simulink model "USV_SAR_GNSS"  (R2026b)
settings: Solver=VariableStepAuto  StopTime=600
undefined symbols (not defined in the file): arrival_dwell_time, arrival_radius, arrival_speed, assistance_duration, battery_capacity_J, battery_initial_soc, battery_return_soc, current_bias_x, current_bias_y, current_change_time, current_estimation_tau, current_x, current_y, drag_r, drag_u, F_max, gnss_bias_x, gnss_bias_y, gnss_loss_enabled, gnss_loss_end, gnss_loss_start, gnss_position_sigma, gnss_sample_time, home_x, home_y, inertia_z, initial_heading, initial_x, initial_y, integral_activation_radius, K_aw, K_distance, Kd_heading, Ki_position, Ki_u, Kp_heading, Kp_u, M_max, mass_usv, mob_contact_loss_enabled, mob_contact_loss_end, mob_contact_loss_start, mob_drift_change_enabled, mob_drift_change_time, mob_drift_factor_after, mob_position_sigma, mob_sensor_sample_time, mob_track_alpha, mob_track_beta, mob_track_max_age, mob_track_sample_time, nav_alpha, nav_beta, nav_max_prediction_time, nav_sample_time, num_waypoints, P_aux, P_thrust_max, P_turn_max, position_integral_limit ... (+6)
libraries: simulink x7
(part 1 of 2)
settings Model: Creator=pablo  LastModifiedBy=pablo

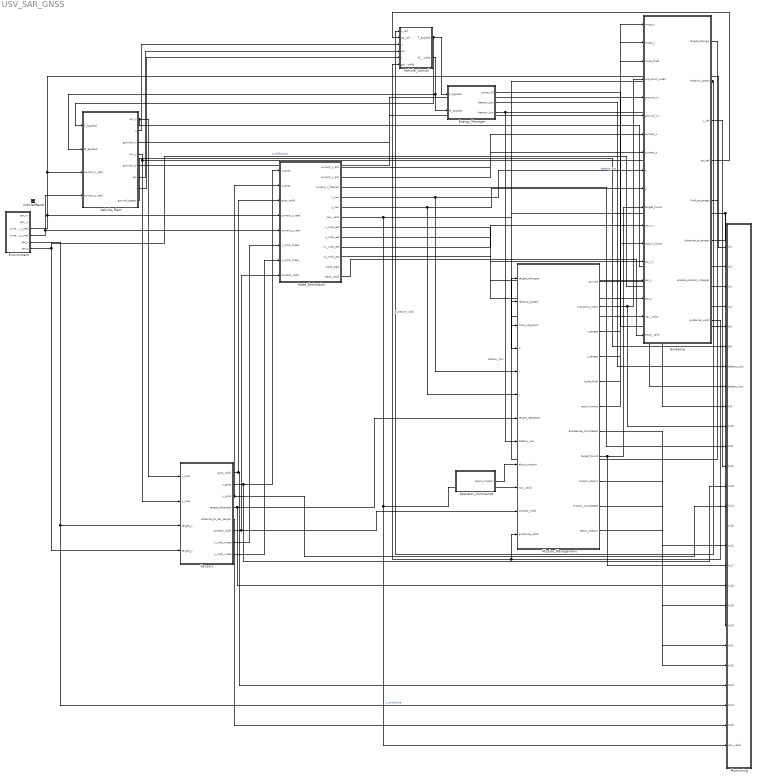
== system USV_SAR_GNSS ==
  Energy_Manager : Subsystem
  Environment : Subsystem
  Guidance : Subsystem
  Mission_Management : Subsystem
  Monitoring : Subsystem
  Operator_Commands : Subsystem
  Sensors : Subsystem
  State_Estimation : Subsystem
  Vehicle_Control : Subsystem
  Vehicle_Plant : Subsystem
  untitledPanel : Subsystem  Tag=HiddenForWebPanel  IsWebBlockPanel=on
  wires:
  Environment/6(sar_y) -> Monitoring/3(In3), Sensors/4(target_y)  "y_mob_true"
  Environment/5(sar_x) -> Monitoring/24(In24), Sensors/3(target_x)  "x_mob_true"
  Environment/4(current_y_real) -> State_Estimation/5(current_y_real), Vehicle_Plant/4(current_y_real)
  Environment/3(current_x_real) -> Monitoring/1(In1), Vehicle_Plant/3(current_x_real), State_Estimation/4(current_x_real)
  Vehicle_Plant/1(usv_x) -> Monitoring/2(In2), Sensors/1(x_true)
  State_Estimation/6(nav_valid) -> Mission_Management/10(nav_valid), Monitoring/26(nav_valid), Guidance/17(nav_valid)
  Vehicle_Plant/2(u) -> Vehicle_Control/3(u)
  Vehicle_Plant/3(ground_vx) -> Guidance/5(ground_vx)
  Vehicle_Plant/4(usv_y) -> Monitoring/4(In4), Sensors/2(y_true)
  Vehicle_Plant/5(ground_vy) -> Guidance/6(ground_vy)
  Vehicle_Plant/6(psi) -> Vehicle_Control/4(psi)
  Energy_Manager/2(battery_soc) -> Monitoring/7(battery_soc)  "battery_soc"
  Vehicle_Plant/7(r) -> Vehicle_Control/5(r)
  Sensors/6(contact_valid) -> Mission_Management/11(contact_valid), State_Estimation/8(contact_valid)
  Vehicle_Plant/8(ground_speed) -> Monitoring/6(In6)
  Sensors/1(gnss_valid) -> Monitoring/23(In23), State_Estimation/3(gnss_valid)
  Operator_Commands/1(abort_mission) -> Mission_Management/9(abort_mission)
  State_Estimation/7(x_mob_est) -> Guidance/15(sar_x)
  Sensors/2(x_gnss) -> Monitoring/13(In13), State_Estimation/1(x_gnss)
  State_Estimation/10(vy_mob_est) -> Guidance/14(sar_vy)
  Sensors/3(y_gnss) -> Monitoring/14(In14), State_Estimation/2(y_gnss)
  State_Estimation/1(current_x_est) -> Guidance/7(current_x)
  Sensors/4(target_detected) -> Monitoring/18(In18), Mission_Management/7(target_detected)
  State_Estimation/4(x_nav) -> Guidance/9(x), Mission_Management/5(x)
  Sensors/5(distance_to_sar_target) -> Monitoring/25(In25)
  Sensors/7(x_mob_meas) -> State_Estimation/6(x_mob_meas)
  Sensors/8(y_mob_meas) -> State_Estimation/7(y_mob_meas)
  State_Estimation/2(current_y_est) -> Guidance/8(current_y)
  State_Estimation/3(current_x_filtered) -> Monitoring/11(In11)
  State_Estimation/5(y_nav) -> Guidance/10(y), Mission_Management/6(y)
  State_Estimation/8(y_mob_est) -> Guidance/16(sar_y)
  State_Estimation/9(vx_mob_est) -> Guidance/12(sar_vx)
  Mission_Management/2(waypoint_index) -> Monitoring/10(In10), Guidance/4(waypoint_index)
  Vehicle_Control/1(F_applied) -> Vehicle_Plant/1(F_applied), Energy_Manager/1(F_applied)
  Vehicle_Control/2(M_applied) -> Vehicle_Plant/2(M_applied), Energy_Manager/2(M_applied)
  Energy_Manager/3(battery_low) -> Monitoring/8(battery_low), Mission_Management/8(battery_low)  "battery_low"
  Energy_Manager/1(power_W) -> Monitoring/5(In5)
  Mission_Management/1(arrived) -> Monitoring/9(In9)
  Mission_Management/3(x_target) -> Guidance/1(route_x)
  Guidance/6(distance_to_target) -> Monitoring/20(In20), Mission_Management/4(d)
  Guidance/2(relative_speed) -> Monitoring/12(In12), Mission_Management/2(relative_speed)
  Mission_Management/4(y_target) -> Guidance/2(route_y)
  Mission_Management/5(route_final) -> Guidance/3(route_final)
  Mission_Management/6(return_home) -> Guidance/13(return_home)
  Mission_Management/7(assistance_completed) -> Monitoring/16(In16)
  Guidance/3(u_ref) -> Vehicle_Control/1(u_ref)
  Mission_Management/8(target_found) -> Monitoring/17(In17), Guidance/11(target_found)
  Mission_Management/9(mission_status) -> Monitoring/19(In19)
  Mission_Management/10(mission_completed) -> Monitoring/21(In21)
  Mission_Management/11(return_reason) -> Monitoring/22(In22)
  Guidance/5(hold_at_target) -> Mission_Management/3(final_waypoint)
  Guidance/1(target_change) -> Mission_Management/1(target_changed)
  Guidance/4(psi_ref) -> Vehicle_Control/2(psi_ref)
  State_Estimation/12(track_valid) -> Guidance/18(track_valid)
  Guidance/8(guidance_valid) -> Mission_Management/12(guidance_valid), Vehicle_Control/6(guidance_valid)  "guidance_valid"

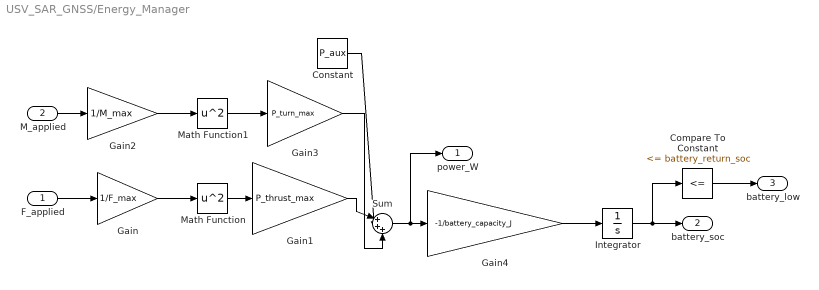
== system USV_SAR_GNSS/Energy_Manager ==
  F_applied : Inport
  M_applied : Inport  Port=2
  Compare To Constant : simulink/Logic and Bit Operations/Compare To Constant  relop=<=  const=battery_return_soc  OutDataTypeStr=boolean
  Constant : Constant  Value=P_aux
  Gain : Gain  Gain=1/F_max
  Gain1 : Gain  Gain=P_thrust_max
  Gain2 : Gain  Gain=1/M_max
  Gain3 : Gain  Gain=P_turn_max
  Gain4 : Gain  Gain=-1/battery_capacity_J
  Integrator : Integrator  InitialCondition=battery_initial_soc  LimitOutput=on  UpperSaturationLimit=1  LowerSaturationLimit=0
  Math Function : Math  Operator=square
  Math Function1 : Math  Operator=square
  Sum : Sum  Inputs=|+++
  power_W : Outport
  battery_soc : Outport  Port=2
  battery_low : Outport  Port=3
  wires:
  Gain2/1 -> Math Function1/1
  M_applied/1 -> Gain2/1
  F_applied/1 -> Gain/1
  Math Function1/1 -> Gain3/1
  Gain/1 -> Math Function/1
  Math Function/1 -> Gain1/1
  Constant/1 -> Sum/2
  Gain3/1 -> Sum/3
  Gain1/1 -> Sum/1
  Sum/1 -> power_W/1, Gain4/1
  Gain4/1 -> Integrator/1
  Integrator/1 -> battery_soc/1, Compare To Constant/1
  Compare To Constant/1 -> battery_low/1

== system USV_SAR_GNSS/Environment ==
  Current_Environment : Subsystem
  SAR_Target_Motion : Subsystem
  sar_vx : Outport
  sar_vy : Outport  Port=2
  current_x_real : Outport  Port=3
  current_y_real : Outport  Port=4
  sar_x : Outport  Port=5
  sar_y : Outport  Port=6
  wires:
  Current_Environment/2(current_y_real) -> SAR_Target_Motion/2(current_y_real), current_y_real/1
  Current_Environment/1(current_x_real) -> current_x_real/1, SAR_Target_Motion/1(current_x_real)
  SAR_Target_Motion/3(sar_vx) -> sar_vx/1  "vx_mob_true"
  SAR_Target_Motion/1(sar_x) -> sar_x/1
  SAR_Target_Motion/4(sar_vy) -> sar_vy/1  "vy_mob_true"
  SAR_Target_Motion/2(sar_y) -> sar_y/1

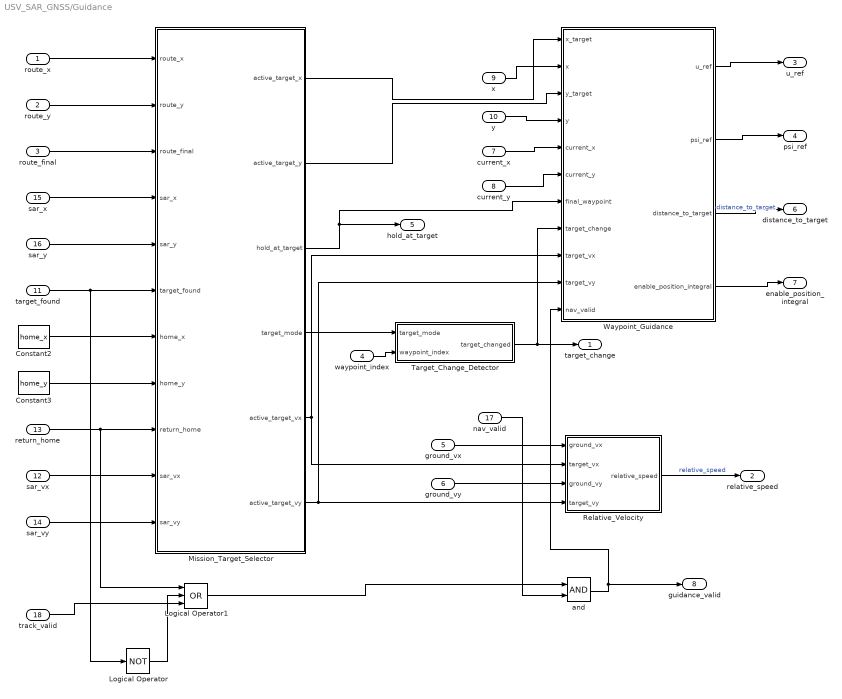
== system USV_SAR_GNSS/Guidance ==
  route_x : Inport
  route_y : Inport  Port=2
  route_final : Inport  Port=3
  waypoint_index : Inport  Port=4
  ground_vx : Inport  Port=5
  ground_vy : Inport  Port=6
  current_x : Inport  Port=7
  current_y : Inport  Port=8
  x : Inport  Port=9
  y : Inport  Port=10
  target_found : Inport  Port=11
  sar_vx : Inport  Port=12
  return_home : Inport  Port=13
  sar_vy : Inport  Port=14
  sar_x : Inport  Port=15
  sar_y : Inport  Port=16
  nav_valid : Inport  Port=17
  track_valid : Inport  Port=18
  Constant2 : Constant  Value=home_x
  Constant3 : Constant  Value=home_y
  Logical Operator : Logic  Operator=NOT  AllPortsSameDT=off  OutDataTypeStr=boolean
  Logical Operator1 : Logic  Operator=OR  Inputs=3  AllPortsSameDT=off  OutDataTypeStr=boolean
  Mission_Target_Selector : Subsystem
  Relative_Velocity : Subsystem
  Target_Change_Detector : Subsystem
  Waypoint_Guidance : Subsystem
  and : Logic  AllPortsSameDT=off  OutDataTypeStr=boolean
  target_change : Outport
  relative_speed : Outport  Port=2
  u_ref : Outport  Port=3
  psi_ref : Outport  Port=4
  hold_at_target : Outport  Port=5
  distance_to_target : Outport  Port=6
  enable_position_integral : Outport  Port=7
  guidance_valid : Outport  Port=8
  wires:
  Waypoint_Guidance/1(u_ref) -> u_ref/1
  Constant3/1 -> Mission_Target_Selector/8(home_y)
  ground_vx/1 -> Relative_Velocity/1(ground_vx)
  Constant2/1 -> Mission_Target_Selector/7(home_x)
  Waypoint_Guidance/3(distance_to_target) -> distance_to_target/1  "distance_to_target"
  Relative_Velocity/1(relative_speed) -> relative_speed/1  "relative_speed"
  route_x/1 -> Mission_Target_Selector/1(route_x)
  route_y/1 -> Mission_Target_Selector/2(route_y)
  Waypoint_Guidance/2(psi_ref) -> psi_ref/1
  target_found/1 -> Logical Operator/1, Mission_Target_Selector/6(target_found)
  sar_x/1 -> Mission_Target_Selector/4(sar_x)
  route_final/1 -> Mission_Target_Selector/3(route_final)
  sar_y/1 -> Mission_Target_Selector/5(sar_y)
  return_home/1 -> Logical Operator1/1, Mission_Target_Selector/9(return_home)
  sar_vx/1 -> Mission_Target_Selector/10(sar_vx)
  Mission_Target_Selector/1(active_target_x) -> Waypoint_Guidance/1(x_target)
  sar_vy/1 -> Mission_Target_Selector/11(sar_vy)
  ground_vy/1 -> Relative_Velocity/3(ground_vy)
  y/1 -> Waypoint_Guidance/4(y)
  Mission_Target_Selector/2(active_target_y) -> Waypoint_Guidance/3(y_target)
  Mission_Target_Selector/3(hold_at_target) -> Waypoint_Guidance/7(final_waypoint), hold_at_target/1
  Mission_Target_Selector/4(target_mode) -> Target_Change_Detector/1(target_mode)
  Mission_Target_Selector/5(active_target_vx) -> Waypoint_Guidance/9(target_vx), Relative_Velocity/2(target_vx)
  Mission_Target_Selector/6(active_target_vy) -> Waypoint_Guidance/10(target_vy), Relative_Velocity/4(target_vy)
  waypoint_index/1 -> Target_Change_Detector/2(waypoint_index)
  x/1 -> Waypoint_Guidance/2(x)
  Waypoint_Guidance/4(enable_position_integral) -> enable_position_integral/1
  current_x/1 -> Waypoint_Guidance/5(current_x)
  current_y/1 -> Waypoint_Guidance/6(current_y)
  Target_Change_Detector/1(target_changed) -> Waypoint_Guidance/8(target_change), target_change/1
  nav_valid/1 -> and/2
  track_valid/1 -> Logical Operator1/3
  Logical Operator/1 -> Logical Operator1/2
  Logical Operator1/1 -> and/1
  and/1 -> Waypoint_Guidance/11(nav_valid), guidance_valid/1

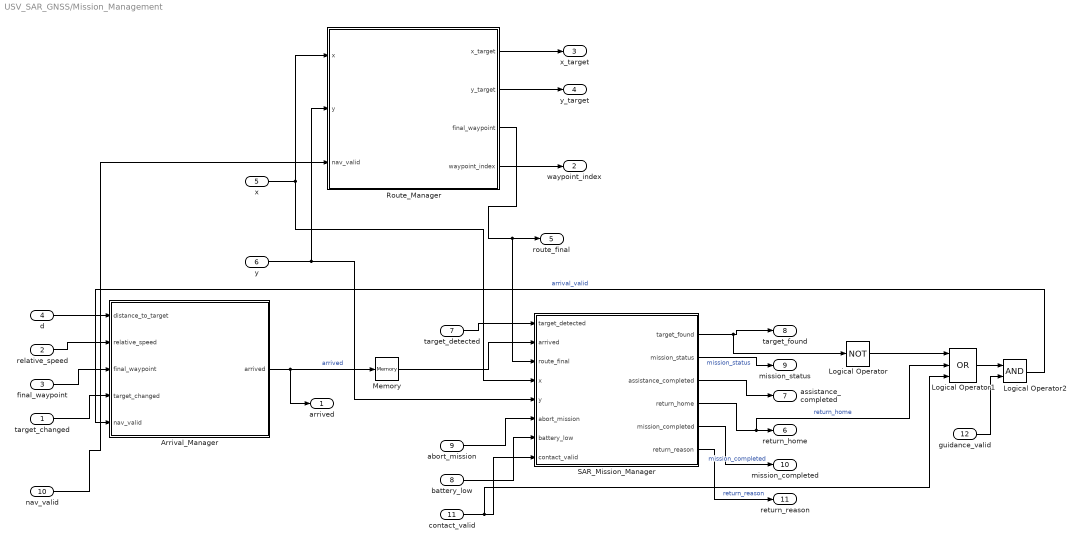
== system USV_SAR_GNSS/Mission_Management ==
  target_changed : Inport
  relative_speed : Inport  Port=2
  final_waypoint : Inport  Port=3
  d : Inport  Port=4
  x : Inport  Port=5
  y : Inport  Port=6
  target_detected : Inport  Port=7
  battery_low : Inport  Port=8
  abort_mission : Inport  Port=9
  nav_valid : Inport  Port=10
  contact_valid : Inport  Port=11
  guidance_valid : Inport  Port=12
  Arrival_Manager : Stateflow chart  TreatAsAtomicUnit=on
  Logical Operator : Logic  Operator=NOT  AllPortsSameDT=off  OutDataTypeStr=boolean
  Logical Operator1 : Logic  Operator=OR  Inputs=3  AllPortsSameDT=off  OutDataTypeStr=boolean
  Logical Operator2 : Logic  AllPortsSameDT=off  OutDataTypeStr=boolean
  Memory : Memory
  Route_Manager : Stateflow chart  TreatAsAtomicUnit=on
  SAR_Mission_Manager : Stateflow chart  TreatAsAtomicUnit=on
  arrived : Outport
  waypoint_index : Outport  Port=2
  x_target : Outport  Port=3
  y_target : Outport  Port=4
  route_final : Outport  Port=5
  return_home : Outport  Port=6
  assistance_completed : Outport  Port=7
  target_found : Outport  Port=8
  mission_status : Outport  Port=9
  mission_completed : Outport  Port=10
  return_reason : Outport  Port=11
  wires:
  d/1 -> Arrival_Manager/1(distance_to_target)
  SAR_Mission_Manager/6(return_reason) -> return_reason/1  "return_reason"
  target_changed/1 -> Arrival_Manager/4(target_changed)
  final_waypoint/1 -> Arrival_Manager/3(final_waypoint)
  SAR_Mission_Manager/3(assistance_completed) -> assistance_completed/1
  abort_mission/1 -> SAR_Mission_Manager/6(abort_mission)
  relative_speed/1 -> Arrival_Manager/2(relative_speed)
  Arrival_Manager/1(arrived) -> arrived/1, Memory/1  "arrived"
  y/1 -> SAR_Mission_Manager/5(y), Route_Manager/2(y)
  x/1 -> SAR_Mission_Manager/4(x), Route_Manager/1(x)
  Route_Manager/1(x_target) -> x_target/1
  Route_Manager/2(y_target) -> y_target/1
  Route_Manager/3(final_waypoint) -> SAR_Mission_Manager/3(route_final), route_final/1
  Route_Manager/4(waypoint_index) -> waypoint_index/1
  target_detected/1 -> SAR_Mission_Manager/1(target_detected)
  Memory/1 -> SAR_Mission_Manager/2(arrived)
  battery_low/1 -> SAR_Mission_Manager/7(battery_low)
  SAR_Mission_Manager/1(target_found) -> Logical Operator/1, target_found/1
  SAR_Mission_Manager/2(mission_status) -> mission_status/1  "mission_status"
  SAR_Mission_Manager/4(return_home) -> Logical Operator1/2, return_home/1  "return_home"
  SAR_Mission_Manager/5(mission_completed) -> mission_completed/1  "mission_completed"
  nav_valid/1 -> Route_Manager/3(nav_valid)
  contact_valid/1 -> Logical Operator1/3, SAR_Mission_Manager/8(contact_valid)
  Logical Operator/1 -> Logical Operator1/1
  Logical Operator1/1 -> Logical Operator2/1
  guidance_valid/1 -> Logical Operator2/2
  Logical Operator2/1 -> Arrival_Manager/5(nav_valid)  "arrival_valid"

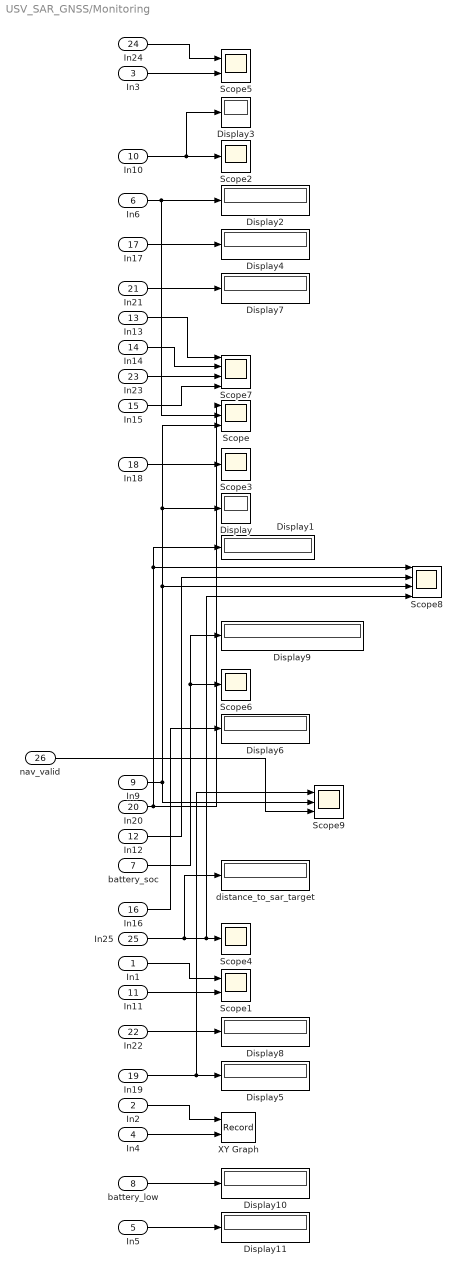
== system USV_SAR_GNSS/Monitoring ==
  In1 : Inport
  In2 : Inport  Port=2
  In3 : Inport  Port=3
  In4 : Inport  Port=4
  In5 : Inport  Port=5
  In6 : Inport  Port=6
  battery_soc : Inport  Port=7
  battery_low : Inport  Port=8
  In9 : Inport  Port=9
  In10 : Inport  Port=10
  In11 : Inport  Port=11
  In12 : Inport  Port=12
  In13 : Inport  Port=13
  In14 : Inport  Port=14
  In15 : Inport  Port=15
  In16 : Inport  Port=16
  In17 : Inport  Port=17
  In18 : Inport  Port=18
  In19 : Inport  Port=19
  In20 : Inport  Port=20
  In21 : Inport  Port=21
  In22 : Inport  Port=22
  In23 : Inport  Port=23
  In24 : Inport  Port=24
  In25 : Inport  Port=25
  nav_valid : Inport  Port=26
  Display{,1..11} (12 alike) : Display
  Scope : Scope  NumInputPorts=3
      settings: ActiveDisplayYMinimum=-3.9141031212329302  ActiveDisplayYMaximum=39.009126348576444
  Scope1 : Scope  NumInputPorts=2
      settings: ActiveDisplayYMinimum=-0.25  ActiveDisplayYMaximum=0.25
  Scope{2..4,6} (4 alike) : Scope
      Scope2 settings: ActiveDisplayYMinimum=-8.8280515458215767  ActiveDisplayYMaximum=9.3125380233394175  DataLoggingVariableName=ScopeData2
      Scope3 settings: ActiveDisplayYMinimum=0.096949603045415472  ActiveDisplayYMaximum=1.0318774717483707  DataLoggingVariableName=ScopeData3
      Scope4 settings: ActiveDisplayYMinimum=-1.9004946435428702E+6  ActiveDisplayYMaximum=1.5322246928084393E+6  DataLoggingVariableName=ScopeData4
      Scope6 settings: ActiveDisplayYMinimum=0.9  ActiveDisplayYMaximum=1.1  DataLoggingVariableName=ScopeData6
  Scope5 : Scope  NumInputPorts=2
      settings: ActiveDisplayYMinimum=-44.000000000000014  ActiveDisplayYMaximum=76.000000000000028  DataLoggingVariableName=ScopeData5
  Scope7 : Scope  NumInputPorts=4
      settings: ActiveDisplayYMinimum=-12.806626439493318  ActiveDisplayYMaximum=22.267972808748297  DataLoggingVariableName=ScopeData7
  Scope8 : Scope  NumInputPorts=4
      settings: ActiveDisplayYMinimum=-3.0987987776116084  ActiveDisplayYMaximum=12.732026530654965  DataLoggingVariableName=ScopeData8
  Scope9 : Scope  NumInputPorts=3
      settings: ActiveDisplayYMinimum=-0.62499999999999989  ActiveDisplayYMaximum=5.625  DataLoggingVariableName=ScopeData9
  XY Graph : Record  NumPorts=2.0  FileSettingsInternal="{\"entries\":[{\"content\":{\"excelSettings\":{\"content\":{},\"type\":\"Streamout.ExcelSettings\"},\"parquetSettings\":{\"content\":{},\"type\":\"Streamout.ParquetSettings\"}},\"type\":\"Streamout.FileSettingStorage\",\"uuid\":\"\"}],\"packageUris\":[\"http:\\/\\/schema.mathworks.com\\/mf0\\/streamout_blocks\\/R2020a\"],\"version\":\"1.0\"}"  FrameSettings=[0, 0]  Layout=[1 1]  SignalsInternal="{\"entries\":[{\"content\":{\"signals\":[{\"content\":{\"blockPath\":[],\"dimensions\":[1],\"domain\":\"\",\"lineColor\":\"#7e2f8e\",\"lineWidth\":2,\"plots\":[ 1 ],\"port\":1,\"sid\":[\"\"],\"signalID\":1,\"signalName\":\"In2\"},\"type\":\"RecordBlkView.Signal\",\"uuid\":\"\"},{\"content\":{\"blockPath\":[],\"dimensions\":[1],\"domain\":\"\",\"lineColor\":\"#77ac30\",\"lineWidth\":2,\"plots\":[ 1 ],\"port\":2,\"sid\":[\"\"],\"signalID\":2,\"signalName\":\"In4\"},\"type\":\"RecordBlkView.Signal\",\"uuid\":\"\"}]},\"type\":\"RecordBlkView.InputSignals\",\"uuid\":\"\"}],\"packageUris\":[\"http:\\/\\/schema.mathworks.com\\/mf0\\/streamout_blocks\\/R2020a\"],\"version\":\"1.0\"}"  VisualizationBindings="{\"xyplotplugin\":{\"info\":[{\"series\":[{\"bindingParametersList\":[{\"parameter\":\"X-Axis\",\"signalID\":1,\"signalName\":\"In2\"},{\"parameter\":\"Y-Axis\",\"signalID\":2,\"signalName\":\"In4\"}],\"seriesID\":0}],\"subplotID\":1}]}}"  CompatibilityTag=XY
  distance_to_sar_target : Display
  wires:
  In22/1 -> Display8/1
  In6/1 -> Scope/2, Display2/1
  In14/1 -> Scope7/2
  In5/1 -> Display11/1
  In21/1 -> Display7/1
  In13/1 -> Scope7/1
  In1/1 -> Scope1/1
  In25/1 -> Scope8/4, Scope4/1, distance_to_sar_target/1
  In9/1 -> Display/1, Scope/3, Scope8/3, Scope9/2
  In17/1 -> Display4/1
  In2/1 -> XY Graph/1
  In18/1 -> Scope3/1
  In10/1 -> Scope2/1, Display3/1
  In19/1 -> Scope9/1, Display5/1
  In11/1 -> Scope1/2
  In3/1 -> Scope5/2
  battery_low/1 -> Display10/1
  In16/1 -> Display6/1
  In24/1 -> Scope5/1
  battery_soc/1 -> Display9/1, Scope6/1
  In15/1 -> Scope7/4
  In23/1 -> Scope7/3
  In4/1 -> XY Graph/2
  In12/1 -> Scope8/2
  In20/1 -> Display1/1, Scope8/1, Scope/1
  nav_valid/1 -> Scope9/3

== system USV_SAR_GNSS/Operator_Commands ==
  Cancel_Release_Step : Step  Time=11  FinalValue=0  SampleTime=0
  Data Type Conversion : DataTypeConversion  OutDataTypeStr=boolean  SaturateOnIntegerOverflow=off  RndMeth=Floor
  Step : Step  Time=100  FinalValue=0  SampleTime=0
  Sum : Sum  Inputs=|+-
  abort_mission : Outport
  wires:
  Step/1 -> Sum/1
  Data Type Conversion/1 -> abort_mission/1  "abort_mission"
  Sum/1 -> Data Type Conversion/1
  Cancel_Release_Step/1 -> Sum/2

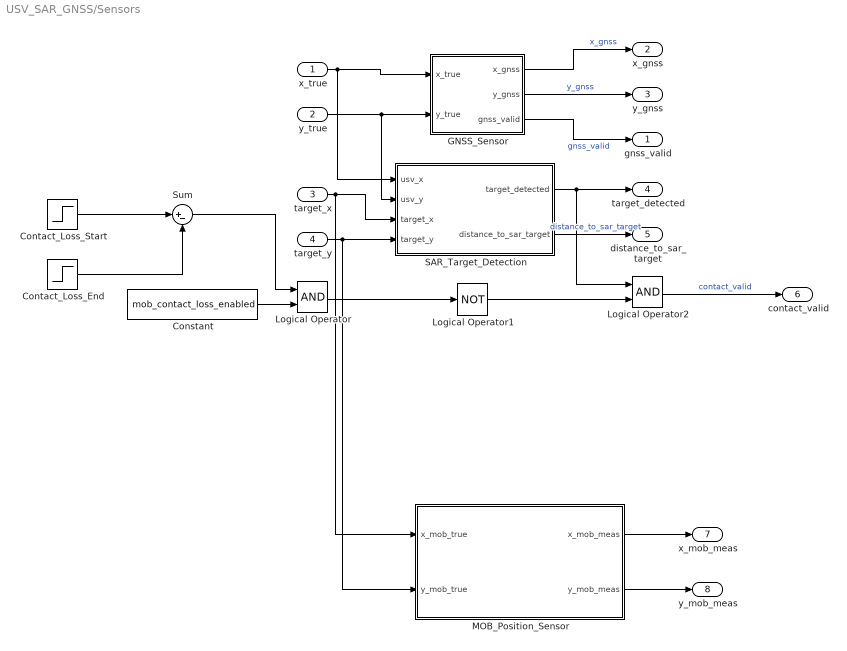
== system USV_SAR_GNSS/Sensors ==
  x_true : Inport
  y_true : Inport  Port=2
  target_x : Inport  Port=3
  target_y : Inport  Port=4
  Constant : Constant  Value=mob_contact_loss_enabled
  Contact_Loss_End : Step  Time=mob_contact_loss_end  SampleTime=0
  Contact_Loss_Start : Step  Time=mob_contact_loss_start  SampleTime=0
  GNSS_Sensor : Subsystem
  Logical Operator : Logic  AllPortsSameDT=off  OutDataTypeStr=boolean
  Logical Operator1 : Logic  Operator=NOT  AllPortsSameDT=off  OutDataTypeStr=boolean
  Logical Operator2 : Logic  AllPortsSameDT=off  OutDataTypeStr=boolean
  MOB_Position_Sensor : Subsystem
  SAR_Target_Detection : Subsystem
  Sum : Sum  Inputs=|+-
  gnss_valid : Outport
  x_gnss : Outport  Port=2
  y_gnss : Outport  Port=3
  target_detected : Outport  Port=4
  distance_to_sar_target : Outport  Port=5
  contact_valid : Outport  Port=6
  x_mob_meas : Outport  Port=7
  y_mob_meas : Outport  Port=8
  wires:
  Constant/1 -> Logical Operator/2
  Sum/1 -> Logical Operator/1
  Contact_Loss_End/1 -> Sum/2
  Contact_Loss_Start/1 -> Sum/1
  target_y/1 -> MOB_Position_Sensor/2(y_mob_true), SAR_Target_Detection/4(target_y)
  target_x/1 -> MOB_Position_Sensor/1(x_mob_true), SAR_Target_Detection/3(target_x)
  y_true/1 -> GNSS_Sensor/2(y_true), SAR_Target_Detection/2(usv_y)
  x_true/1 -> GNSS_Sensor/1(x_true), SAR_Target_Detection/1(usv_x)
  Logical Operator/1 -> Logical Operator1/1
  GNSS_Sensor/1(x_gnss) -> x_gnss/1  "x_gnss"
  GNSS_Sensor/2(y_gnss) -> y_gnss/1  "y_gnss"
  Logical Operator1/1 -> Logical Operator2/2
  GNSS_Sensor/3(gnss_valid) -> gnss_valid/1  "gnss_valid"
  SAR_Target_Detection/1(target_detected) -> Logical Operator2/1, target_detected/1
  SAR_Target_Detection/2(distance_to_sar_target) -> distance_to_sar_target/1  "distance_to_sar_target"
  Logical Operator2/1 -> contact_valid/1  "contact_valid"
  MOB_Position_Sensor/1(x_mob_meas) -> x_mob_meas/1
  MOB_Position_Sensor/2(y_mob_meas) -> y_mob_meas/1

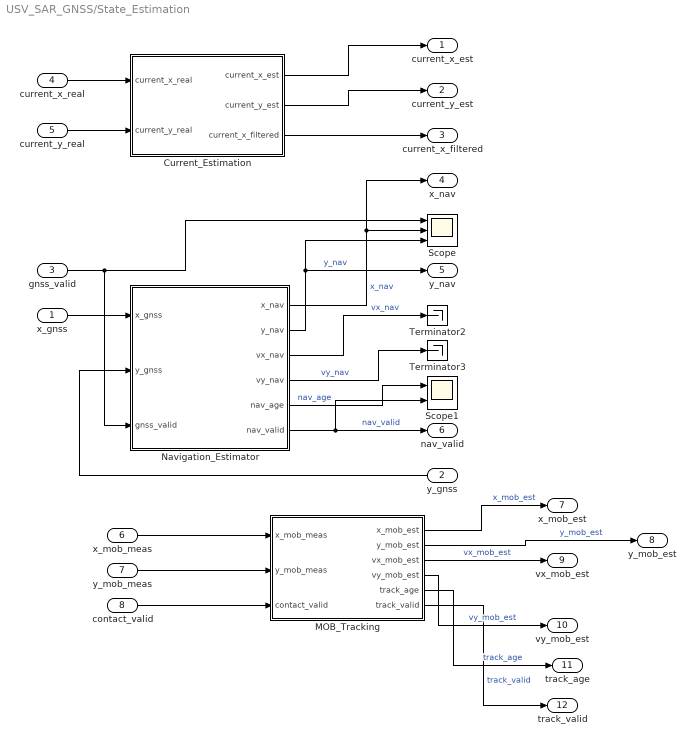
== system USV_SAR_GNSS/State_Estimation ==
  x_gnss : Inport
  y_gnss : Inport  Port=2
  gnss_valid : Inport  Port=3
  current_x_real : Inport  Port=4
  current_y_real : Inport  Port=5
  x_mob_meas : Inport  Port=6
  y_mob_meas : Inport  Port=7
  contact_valid : Inport  Port=8
  Current_Estimation : Subsystem
  MOB_Tracking : Subsystem
  Navigation_Estimator : Subsystem
  Scope : Scope  NumInputPorts=3
      settings: ActiveDisplayYMinimum=-0.26944529643328874  ActiveDisplayYMaximum=48.836838243913448  DataLoggingVariableName=ScopeData10
  Scope1 : Scope  NumInputPorts=2
      settings: ActiveDisplayYMinimum=-2.6125000000000029  ActiveDisplayYMaximum=23.512500000000031  DataLoggingVariableName=ScopeData11
  Terminator2 : Terminator
  Terminator3 : Terminator
  current_x_est : Outport
  current_y_est : Outport  Port=2
  current_x_filtered : Outport  Port=3
  x_nav : Outport  Port=4
  y_nav : Outport  Port=5
  nav_valid : Outport  Port=6
  x_mob_est : Outport  Port=7
  y_mob_est : Outport  Port=8
  vx_mob_est : Outport  Port=9
  vy_mob_est : Outport  Port=10
  track_age : Outport  Port=11
  track_valid : Outport  Port=12
  wires:
  x_gnss/1 -> Navigation_Estimator/1(x_gnss)
  current_x_real/1 -> Current_Estimation/1(current_x_real)
  Current_Estimation/3(current_x_filtered) -> current_x_filtered/1
  Current_Estimation/1(current_x_est) -> current_x_est/1
  gnss_valid/1 -> Scope/1, Navigation_Estimator/3(gnss_valid)
  current_y_real/1 -> Current_Estimation/2(current_y_real)
  Current_Estimation/2(current_y_est) -> current_y_est/1
  Navigation_Estimator/1(x_nav) -> Scope/2, x_nav/1  "x_nav"
  Navigation_Estimator/2(y_nav) -> Scope/3, y_nav/1  "y_nav"
  Navigation_Estimator/3(vx_nav) -> Terminator2/1  "vx_nav"
  Navigation_Estimator/4(vy_nav) -> Terminator3/1  "vy_nav"
  Navigation_Estimator/5(nav_age) -> Scope1/1  "nav_age"
  Navigation_Estimator/6(nav_valid) -> nav_valid/1, Scope1/2  "nav_valid"
  y_gnss/1 -> Navigation_Estimator/2(y_gnss)
  x_mob_meas/1 -> MOB_Tracking/1(x_mob_meas)
  contact_valid/1 -> MOB_Tracking/3(contact_valid)
  y_mob_meas/1 -> MOB_Tracking/2(y_mob_meas)
  MOB_Tracking/1(x_mob_est) -> x_mob_est/1  "x_mob_est"
  MOB_Tracking/2(y_mob_est) -> y_mob_est/1  "y_mob_est"
  MOB_Tracking/3(vx_mob_est) -> vx_mob_est/1  "vx_mob_est"
  MOB_Tracking/4(vy_mob_est) -> vy_mob_est/1  "vy_mob_est"
  MOB_Tracking/5(track_age) -> track_age/1  "track_age"
  MOB_Tracking/6(track_valid) -> track_valid/1  "track_valid"

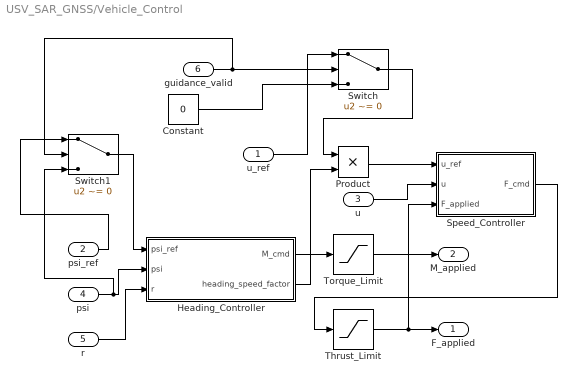
== system USV_SAR_GNSS/Vehicle_Control ==
  u_ref : Inport
  psi_ref : Inport  Port=2
  u : Inport  Port=3
  psi : Inport  Port=4
  r : Inport  Port=5
  guidance_valid : Inport  Port=6
  Constant : Constant  Value=0
  Heading_Controller : Subsystem
  Product : Product
  Speed_Controller : Subsystem
  Switch : Switch  Criteria=u2 ~= 0  SaturateOnIntegerOverflow=off  InputSameDT=off
  Switch1 : Switch  Criteria=u2 ~= 0  SaturateOnIntegerOverflow=off  InputSameDT=off
  Thrust_Limit : Saturate  UpperLimit=F_max  LowerLimit=-F_max
  Torque_Limit : Saturate  UpperLimit=M_max  LowerLimit=-M_max
  F_applied : Outport
  M_applied : Outport  Port=2
  wires:
  psi_ref/1 -> Switch1/1
  psi/1 -> Switch1/3, Heading_Controller/2(psi)
  Heading_Controller/2(heading_speed_factor) -> Product/2
  Product/1 -> Speed_Controller/1(u_ref)
  Heading_Controller/1(M_cmd) -> Torque_Limit/1
  u_ref/1 -> Switch/1
  r/1 -> Heading_Controller/3(r)
  u/1 -> Speed_Controller/2(u)
  Torque_Limit/1 -> M_applied/1
  Thrust_Limit/1 -> Speed_Controller/3(F_applied), F_applied/1
  Speed_Controller/1(F_cmd) -> Thrust_Limit/1
  guidance_valid/1 -> Switch1/2, Switch/2
  Constant/1 -> Switch/3
  Switch/1 -> Product/1
  Switch1/1 -> Heading_Controller/1(psi_ref)

== system USV_SAR_GNSS/Vehicle_Plant ==
  F_applied : Inport
  M_applied : Inport  Port=2
  current_x_real : Inport  Port=3
  current_y_real : Inport  Port=4
  USV_Dynamics : Subsystem
  USV_Kinematics : Subsystem
  usv_x : Outport
  u : Outport  Port=2
  ground_vx : Outport  Port=3
  usv_y : Outport  Port=4
  ground_vy : Outport  Port=5
  psi : Outport  Port=6
  r : Outport  Port=7
  ground_speed : Outport  Port=8
  wires:
  USV_Kinematics/2(y) -> usv_y/1  "usv_y"
  F_applied/1 -> USV_Dynamics/1(F_cmd)
  M_applied/1 -> USV_Dynamics/2(M_cmd)
  USV_Dynamics/1(u) -> USV_Kinematics/1(u), u/1
  USV_Dynamics/2(r) -> r/1, USV_Kinematics/2(r)
  USV_Kinematics/1(x) -> usv_x/1  "usv_x"
  current_x_real/1 -> USV_Kinematics/3(current_x)
  current_y_real/1 -> USV_Kinematics/4(current_y)
  USV_Kinematics/3(psi) -> psi/1
  USV_Kinematics/4(ground_speed) -> ground_speed/1
  USV_Kinematics/5(ground_vx) -> ground_vx/1
  USV_Kinematics/6(ground_vy) -> ground_vy/1

== system USV_SAR_GNSS/untitledPanel ==
  Display12 : DisplayBlock  Tag=HiddenForWebPanel  PanelInfo="{\"height\":39,\"left\":17,\"panelId\":\"panelId-7d76bbda-0191-40eb-92e3-69925966ccdc\",\"top\":17,\"type\":\"panelChild\",\"version\":\"2019b\",\"width\":174,\"zIndex\":1500002}"  LabelPosition=Hide  Transparency=1  GridColor=[0.502, 0.502, 0.502]
  Display13 : DisplayBlock  Tag=HiddenForWebPanel  PanelInfo="{\"height\":39,\"left\":16,\"panelId\":\"panelId-7d76bbda-0191-40eb-92e3-69925966ccdc\",\"top\":70,\"type\":\"panelChild\",\"version\":\"2019b\",\"width\":174,\"zIndex\":1500004}"  LabelPosition=Hide  Transparency=1  GridColor=[0.502, 0.502, 0.502]
  Display14 : DisplayBlock  Tag=HiddenForWebPanel  PanelInfo="{\"height\":39,\"left\":16,\"panelId\":\"panelId-7d76bbda-0191-40eb-92e3-69925966ccdc\",\"top\":119,\"type\":\"panelChild\",\"version\":\"2019b\",\"width\":174,\"zIndex\":1500006}"  LabelPosition=Hide  Transparency=1  GridColor=[0.502, 0.502, 0.502]
  panelInfo : PanelWebBlock  Tag=HiddenForWebPanel  PanelInfo="{\"compacted\":false,\"height\":256,\"isActiveTab\":true,\"left\":1302,\"name\":\"Panel\",\"panelId\":\"panelId-7d76bbda-0191-40eb-92e3-69925966ccdc\",\"tabIndex\":0,\"tabbedSetId\":\"tabbedSet4358925779\",\"top\":159,\"type\":\"panel\",\"version\":\"2019b\",\"visible\":true,\"width\":237,\"zIndex\":1500002}"  PanelSnapshot=<binary blob, 1920 chars, not shown>

== system USV_SAR_GNSS/Environment/Current_Environment ==
  Step : Step  Time=current_change_time  InitialValue=current_x  FinalValue=current_x_after  SampleTime=0
  Step1 : Step  Time=current_change_time  InitialValue=current_y  FinalValue=current_y_after  SampleTime=0
  current_x_real : Outport
  current_y_real : Outport  Port=2
  wires:
  Step/1 -> current_x_real/1
  Step1/1 -> current_y_real/1

== system USV_SAR_GNSS/Environment/SAR_Target_Motion ==
  current_x_real : Inport
  current_y_real : Inport  Port=2
  Integrator : Integrator  InitialCondition=sar_target_x
  Integrator1 : Integrator  InitialCondition=sar_target_y
  Product : Product
  Product1 : Product
  Step : Step  Time=mob_drift_change_time  InitialValue=sar_drift_factor  FinalValue=sar_drift_factor + double(mob_drift_change_enabled)*(mob_drift_factor_after - sar_drift_factor)  SampleTime=0
  sar_x : Outport
  sar_y : Outport  Port=2
  sar_vx : Outport  Port=3
  sar_vy : Outport  Port=4
  wires:
  Integrator1/1 -> sar_y/1
  Integrator/1 -> sar_x/1
  current_y_real/1 -> Product1/1
  current_x_real/1 -> Product/1
  Product1/1 -> sar_vy/1, Integrator1/1
  Step/1 -> Product/2, Product1/2
  Product/1 -> sar_vx/1, Integrator/1

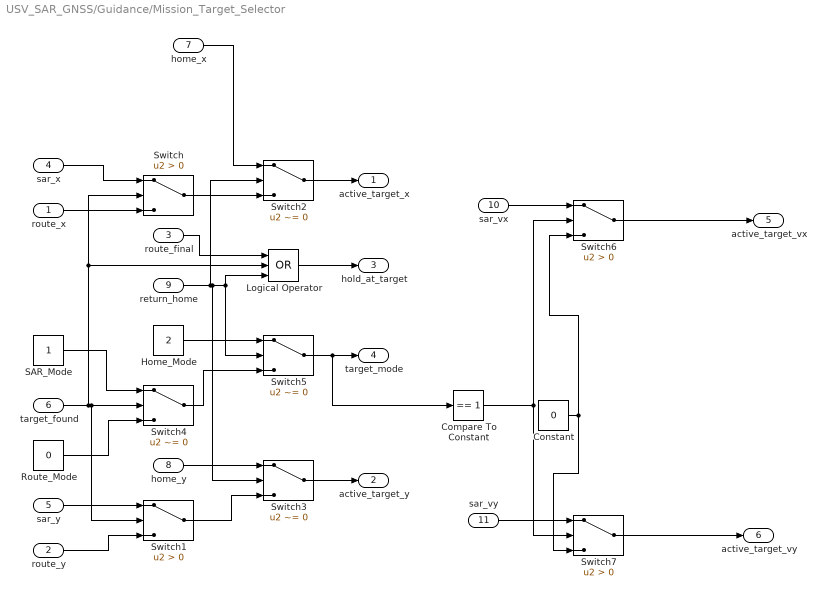
== system USV_SAR_GNSS/Guidance/Mission_Target_Selector ==
  route_x : Inport
  route_y : Inport  Port=2
  route_final : Inport  Port=3
  sar_x : Inport  Port=4
  sar_y : Inport  Port=5
  target_found : Inport  Port=6
  home_x : Inport  Port=7
  home_y : Inport  Port=8
  return_home : Inport  Port=9
  sar_vx : Inport  Port=10
  sar_vy : Inport  Port=11
  Compare To Constant : simulink/Logic and Bit Operations/Compare To Constant  relop===  const=1  OutDataTypeStr=boolean
  Constant : Constant  Value=0
  Home_Mode : Constant  Value=2
  Logical Operator : Logic  Operator=OR  Inputs=3  AllPortsSameDT=off  OutDataTypeStr=boolean
  Route_Mode : Constant  Value=0
  SAR_Mode : Constant
  Switch{,1,6..7} (4 alike) : Switch  Criteria=u2 > Threshold  SaturateOnIntegerOverflow=off  InputSameDT=off
  Switch{2..5} (4 alike) : Switch  Criteria=u2 ~= 0  SaturateOnIntegerOverflow=off  InputSameDT=off
  active_target_x : Outport
  active_target_y : Outport  Port=2
  hold_at_target : Outport  Port=3
  target_mode : Outport  Port=4
  active_target_vx : Outport  Port=5
  active_target_vy : Outport  Port=6
  wires:
  route_final/1 -> Logical Operator/1
  home_x/1 -> Switch2/1
  target_found/1 -> Switch1/2, Switch4/2, Logical Operator/2, Switch/2
  route_y/1 -> Switch1/3
  route_x/1 -> Switch/3
  sar_y/1 -> Switch1/1
  home_y/1 -> Switch3/1
  sar_x/1 -> Switch/1
  Switch4/1 -> Switch5/3
  Route_Mode/1 -> Switch4/3
  SAR_Mode/1 -> Switch4/1
  Switch/1 -> Switch2/3
  return_home/1 -> Logical Operator/3, Switch5/2, Switch3/2, Switch2/2
  Home_Mode/1 -> Switch5/1
  Switch1/1 -> Switch3/3
  Logical Operator/1 -> hold_at_target/1
  Switch2/1 -> active_target_x/1
  Switch5/1 -> Compare To Constant/1, target_mode/1
  Switch3/1 -> active_target_y/1
  Compare To Constant/1 -> Switch6/2, Switch7/2
  sar_vx/1 -> Switch6/1
  sar_vy/1 -> Switch7/1
  Constant/1 -> Switch7/3, Switch6/3
  Switch6/1 -> active_target_vx/1
  Switch7/1 -> active_target_vy/1

== system USV_SAR_GNSS/Guidance/Relative_Velocity ==
  ground_vx : Inport
  target_vx : Inport  Port=2
  ground_vy : Inport  Port=3
  target_vy : Inport  Port=4
  Math Function : Math  Operator=square
  Math Function1 : Math  Operator=square
  Sqrt : Sqrt
  Sum : Sum  Inputs=|+-
  Sum1 : Sum  Inputs=|+-
  Sum2 : Sum  Inputs=|++
  relative_speed : Outport
  wires:
  Sum/1 -> Math Function/1
  ground_vx/1 -> Sum/1
  Math Function1/1 -> Sum2/2
  target_vx/1 -> Sum/2
  ground_vy/1 -> Sum1/1
  Math Function/1 -> Sum2/1
  target_vy/1 -> Sum1/2
  Sum1/1 -> Math Function1/1
  Sum2/1 -> Sqrt/1
  Sqrt/1 -> relative_speed/1

== system USV_SAR_GNSS/Guidance/Target_Change_Detector ==
  target_mode : Inport
  waypoint_index : Inport  Port=2
  Abs : Abs  SaturateOnIntegerOverflow=off
  Abs1 : Abs  SaturateOnIntegerOverflow=off
  Compare To Constant : simulink/Logic and Bit Operations/Compare To Constant  relop=>  const=1e-6  OutDataTypeStr=boolean
  Compare To Constant1 : simulink/Logic and Bit Operations/Compare To Constant  relop=>  const=1e-6  OutDataTypeStr=boolean
  Compare To Constant2 : simulink/Logic and Bit Operations/Compare To Constant  relop===  const=0  OutDataTypeStr=boolean
  Data Type Conversion : DataTypeConversion  OutDataTypeStr=double  SaturateOnIntegerOverflow=off  RndMeth=Floor
  Data Type Conversion1 : DataTypeConversion  OutDataTypeStr=double  SaturateOnIntegerOverflow=off  RndMeth=Floor
  Logical Operator : Logic  Operator=OR  AllPortsSameDT=off  OutDataTypeStr=boolean
  Logical Operator1 : Logic  AllPortsSameDT=off  OutDataTypeStr=boolean
  Memory1 : Memory
  Memory2 : Memory  InitialCondition=1
  Sum : Sum  Inputs=|+-
  Sum1 : Sum  Inputs=|+-
  target_changed : Outport
  wires:
  target_mode/1 -> Data Type Conversion/1
  Abs1/1 -> Compare To Constant1/1
  waypoint_index/1 -> Data Type Conversion1/1
  Sum/1 -> Abs/1
  Memory2/1 -> Sum1/2
  Sum1/1 -> Abs1/1
  Memory1/1 -> Sum/2
  Compare To Constant2/1 -> Logical Operator1/1
  Abs/1 -> Compare To Constant/1
  Logical Operator1/1 -> Logical Operator/2
  Compare To Constant1/1 -> Logical Operator1/2
  Compare To Constant/1 -> Logical Operator/1
  Logical Operator/1 -> target_changed/1
  Data Type Conversion/1 -> Compare To Constant2/1, Memory1/1, Sum/1
  Data Type Conversion1/1 -> Sum1/1, Memory2/1

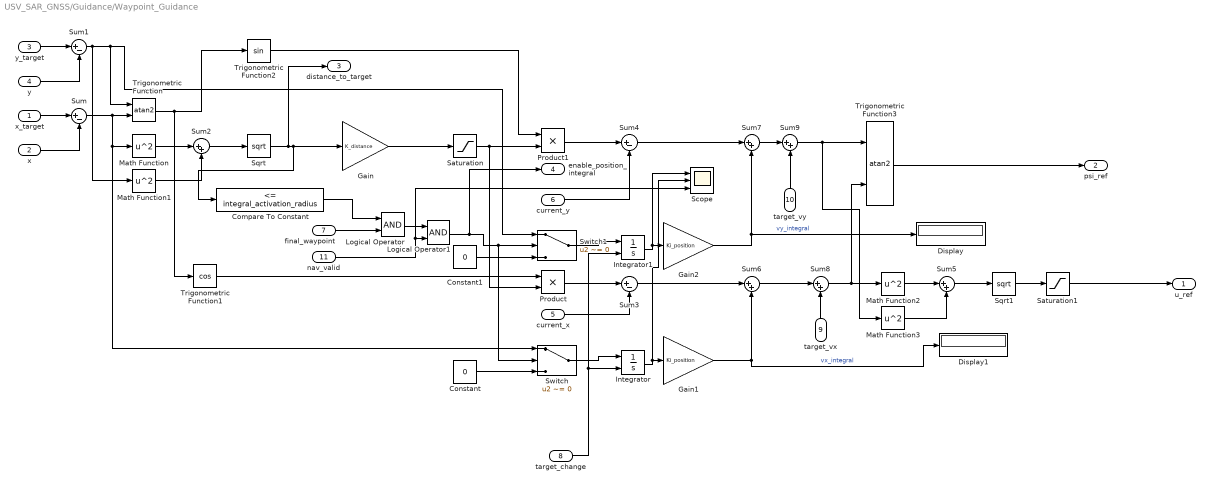
== system USV_SAR_GNSS/Guidance/Waypoint_Guidance ==
  x_target : Inport
  x : Inport  Port=2
  y_target : Inport  Port=3
  y : Inport  Port=4
  current_x : Inport  Port=5
  current_y : Inport  Port=6
  final_waypoint : Inport  Port=7
  target_change : Inport  Port=8
  target_vx : Inport  Port=9
  target_vy : Inport  Port=10
  nav_valid : Inport  Port=11
  Compare To Constant : simulink/Logic and Bit Operations/Compare To Constant  relop=<=  const=integral_activation_radius  OutDataTypeStr=boolean
  Constant : Constant  Value=0
  Constant1 : Constant  Value=0
  Display : Display
  Display1 : Display
  Gain : Gain  Gain=K_distance
  Gain1 : Gain  Gain=Ki_position
  Gain2 : Gain  Gain=Ki_position
  Integrator : Integrator  ExternalReset=rising  LimitOutput=on  UpperSaturationLimit=position_integral_limit  LowerSaturationLimit=-position_integral_limit
  Integrator1 : Integrator  ExternalReset=rising  LimitOutput=on  UpperSaturationLimit=position_integral_limit  LowerSaturationLimit=-position_integral_limit
  Logical Operator : Logic  AllPortsSameDT=off  OutDataTypeStr=boolean
  Logical Operator1 : Logic  AllPortsSameDT=off  OutDataTypeStr=boolean
  Math Function{,1..3} (4 alike) : Math  Operator=square
  Product : Product
  Product1 : Product
  Saturation : Saturate  UpperLimit=u_max  LowerLimit=0
  Saturation1 : Saturate  UpperLimit=u_max  LowerLimit=0
  Scope : Scope  NumInputPorts=3
      settings: ActiveDisplayYMinimum=-5.2833623312781777  ActiveDisplayYMaximum=9.6636815843183044  DataLoggingVariableName=ScopeData12
  Sqrt : Sqrt
  Sqrt1 : Sqrt
  Sum{,1,3..4} (4 alike) : Sum  Inputs=|+-
  Sum{2,5..9} (6 alike) : Sum  Inputs=|++
  Switch : Switch  Criteria=u2 ~= 0  SaturateOnIntegerOverflow=off  InputSameDT=off
  Switch1 : Switch  Criteria=u2 ~= 0  SaturateOnIntegerOverflow=off  InputSameDT=off
  Trigonometric Function : Trigonometry  Operator=atan2
  Trigonometric Function1 : Trigonometry  Operator=cos
  Trigonometric Function2 : Trigonometry
  Trigonometric Function3 : Trigonometry  Operator=atan2
  u_ref : Outport
  psi_ref : Outport  Port=2
  distance_to_target : Outport  Port=3
  enable_position_integral : Outport  Port=4
  wires:
  Product/1 -> Sum3/1
  current_y/1 -> Sum4/2
  x/1 -> Sum/2
  x_target/1 -> Sum/1
  Product1/1 -> Sum4/1
  y/1 -> Sum1/2
  y_target/1 -> Sum1/1
  Switch1/1 -> Integrator1/1
  Trigonometric Function/1 -> Trigonometric Function2/1, Trigonometric Function1/1
  Math Function/1 -> Sum2/1
  Math Function2/1 -> Sum5/1
  Sum2/1 -> Sqrt/1
  Sum/1 -> Switch/1, Math Function/1, Trigonometric Function/2
  Sqrt/1 -> Gain/1, Compare To Constant/1, distance_to_target/1
  Sum1/1 -> Switch1/1, Trigonometric Function/1, Math Function1/1
  Saturation1/1 -> u_ref/1
  Math Function1/1 -> Sum2/2
  Trigonometric Function1/1 -> Product/1
  Switch/1 -> Integrator/1
  Trigonometric Function2/1 -> Product1/1
  Gain/1 -> Saturation/1
  Compare To Constant/1 -> Logical Operator/1
  final_waypoint/1 -> Logical Operator/2
  Constant/1 -> Switch/3
  Saturation/1 -> Product/2, Product1/2
  Sum4/1 -> Sum7/1
  Constant1/1 -> Switch1/3
  current_x/1 -> Sum3/2
  Integrator1/1 -> Scope/1, Gain2/1
  Sum3/1 -> Sum6/1
  Integrator/1 -> Scope/2, Gain1/1
  Gain2/1 -> Sum7/2, Display/1  "vy_integral"
  Gain1/1 -> Sum6/2, Display1/1  "vx_integral"
  Trigonometric Function3/1 -> psi_ref/1
  Sum5/1 -> Sqrt1/1
  Math Function3/1 -> Sum5/2
  Sqrt1/1 -> Saturation1/1
  target_change/1 -> Integrator/2, Integrator1/2
  Sum6/1 -> Sum8/1
  Sum8/1 -> Math Function2/1, Trigonometric Function3/2
  target_vx/1 -> Sum8/2
  Sum7/1 -> Sum9/1
  Sum9/1 -> Math Function3/1, Trigonometric Function3/1
  target_vy/1 -> Sum9/2
  Logical Operator/1 -> Logical Operator1/1
  nav_valid/1 -> Scope/3, Logical Operator1/2
  Logical Operator1/1 -> Switch/2, Switch1/2, enable_position_integral/1

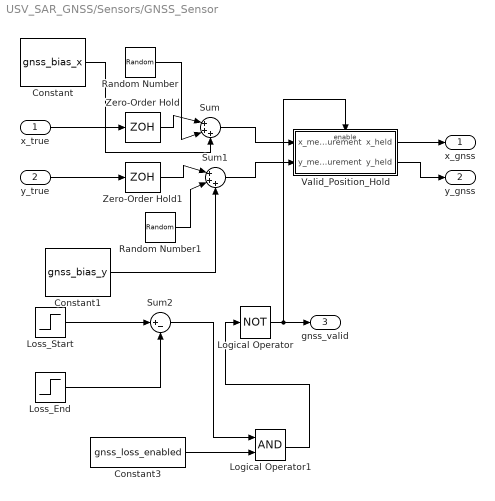
== system USV_SAR_GNSS/Sensors/GNSS_Sensor ==
  x_true : Inport
  y_true : Inport  Port=2
  Constant : Constant  Value=gnss_bias_x
  Constant1 : Constant  Value=gnss_bias_y
  Constant3 : Constant  Value=gnss_loss_enabled
  Logical Operator : Logic  Operator=NOT  AllPortsSameDT=off  OutDataTypeStr=boolean
  Logical Operator1 : Logic  AllPortsSameDT=off  OutDataTypeStr=boolean
  Loss_End : Step  Time=gnss_loss_end  SampleTime=gnss_sample_time
  Loss_Start : Step  Time=gnss_loss_start  SampleTime=gnss_sample_time
  Random Number : RandomNumber  Variance=gnss_position_sigma^2  Seed=11  SampleTime=gnss_sample_time
  Random Number1 : RandomNumber  Variance=gnss_position_sigma^2  Seed=22  SampleTime=gnss_sample_time
  Sum : Sum  Inputs=|+++
  Sum1 : Sum  Inputs=|+++
  Sum2 : Sum  Inputs=|+-
  Valid_Position_Hold : Subsystem  TreatAsAtomicUnit=on
  Zero-Order Hold : ZeroOrderHold  SampleTime=gnss_sample_time
  Zero-Order Hold1 : ZeroOrderHold  SampleTime=gnss_sample_time
  x_gnss : Outport
  y_gnss : Outport  Port=2
  gnss_valid : Outport  Port=3
  wires:
  x_true/1 -> Zero-Order Hold/1
  y_true/1 -> Zero-Order Hold1/1
  Zero-Order Hold/1 -> Sum/1
  Sum/1 -> Valid_Position_Hold/1(x_mesurement)
  Zero-Order Hold1/1 -> Sum1/1
  Sum1/1 -> Valid_Position_Hold/2(y_mesurement)
  Random Number1/1 -> Sum1/2
  Random Number/1 -> Sum/2
  Constant/1 -> Sum/3
  Constant1/1 -> Sum1/3
  Loss_Start/1 -> Sum2/1
  Loss_End/1 -> Sum2/2
  Logical Operator/1 -> gnss_valid/1, Valid_Position_Hold/Enable
  Valid_Position_Hold/1(x_held) -> x_gnss/1
  Valid_Position_Hold/2(y_held) -> y_gnss/1
  Constant3/1 -> Logical Operator1/2
  Sum2/1 -> Logical Operator1/1
  Logical Operator1/1 -> Logical Operator/1

== system USV_SAR_GNSS/Sensors/MOB_Position_Sensor ==
  x_mob_true : Inport
  y_mob_true : Inport  Port=2
  Random Number : RandomNumber  Variance=mob_position_sigma^2  Seed=31  SampleTime=mob_sensor_sample_time
  Random Number1 : RandomNumber  Variance=mob_position_sigma^2  Seed=32  SampleTime=mob_sensor_sample_time
  Sum : Sum  Inputs=|++
  Sum1 : Sum  Inputs=|++
  Zero-Order Hold : ZeroOrderHold  SampleTime=mob_sensor_sample_time
  Zero-Order Hold1 : ZeroOrderHold  SampleTime=mob_sensor_sample_time
  x_mob_meas : Outport
  y_mob_meas : Outport  Port=2
  wires:
  x_mob_true/1 -> Zero-Order Hold/1
  Zero-Order Hold/1 -> Sum/1
  Sum/1 -> x_mob_meas/1  "x_mob_meas"
  Random Number/1 -> Sum/2
  y_mob_true/1 -> Zero-Order Hold1/1
  Zero-Order Hold1/1 -> Sum1/1
  Random Number1/1 -> Sum1/2
  Sum1/1 -> y_mob_meas/1  "y_mob_meas"

== system USV_SAR_GNSS/Sensors/SAR_Target_Detection ==
  usv_x : Inport
  usv_y : Inport  Port=2
  target_x : Inport  Port=3
  target_y : Inport  Port=4
  Compare To Constant : simulink/Logic and Bit Operations/Compare To Constant  relop=<=  const=sar_detection_range  OutDataTypeStr=boolean
  Math Function : Math  Operator=square
  Math Function1 : Math  Operator=square
  Sqrt : Sqrt
  Sum : Sum  Inputs=|+-
  Sum1 : Sum  Inputs=|+-
  Sum2 : Sum  Inputs=|++
  target_detected : Outport
  distance_to_sar_target : Outport  Port=2
  wires:
  Sum1/1 -> Math Function1/1
  Sum/1 -> Math Function/1
  usv_x/1 -> Sum/2
  target_x/1 -> Sum/1
  usv_y/1 -> Sum1/2
  Math Function1/1 -> Sum2/2
  Math Function/1 -> Sum2/1
  Sum2/1 -> Sqrt/1
  target_y/1 -> Sum1/1
  Sqrt/1 -> Compare To Constant/1, distance_to_sar_target/1
  Compare To Constant/1 -> target_detected/1

== system USV_SAR_GNSS/State_Estimation/Current_Estimation ==
  current_x_real : Inport
  current_y_real : Inport  Port=2
  Constant : Constant  Value=current_bias_x
  Constant1 : Constant  Value=current_bias_y
  Gain : Gain  Gain=1/current_estimation_tau
  Gain1 : Gain  Gain=1/current_estimation_tau
  Integrator : Integrator  InitialCondition=current_x
  Integrator1 : Integrator  InitialCondition=current_y
  Sum : Sum  Inputs=|++
  Sum1 : Sum  Inputs=|++
  Sum2 : Sum  Inputs=|+-
  Sum3 : Sum  Inputs=|+-
  current_x_est : Outport
  current_y_est : Outport  Port=2
  current_x_filtered : Outport  Port=3
  wires:
  current_y_real/1 -> Sum3/1
  current_x_real/1 -> Sum2/1
  Gain1/1 -> Integrator1/1
  Sum2/1 -> Gain/1
  Sum3/1 -> Gain1/1
  Gain/1 -> Integrator/1
  Integrator/1 -> Sum/1, current_x_filtered/1, Sum2/2
  Constant/1 -> Sum/2
  Integrator1/1 -> Sum3/2, Sum1/1
  Constant1/1 -> Sum1/2
  Sum/1 -> current_x_est/1
  Sum1/1 -> current_y_est/1

== system USV_SAR_GNSS/State_Estimation/MOB_Tracking ==
  x_mob_meas : Inport
  y_mob_meas : Inport  Port=2
  contact_valid : Inport  Port=3
  MOB_Estimator : MATLAB Function  TreatAsAtomicUnit=on
  x_mob_est : Outport
  y_mob_est : Outport  Port=2
  vx_mob_est : Outport  Port=3
  vy_mob_est : Outport  Port=4
  track_age : Outport  Port=5
  track_valid : Outport  Port=6
  wires:
  x_mob_meas/1 -> MOB_Estimator/1(x_mob_meas)
  y_mob_meas/1 -> MOB_Estimator/2(y_mob_meas)
  contact_valid/1 -> MOB_Estimator/3(contact_valid)
  MOB_Estimator/1(x_mob_est) -> x_mob_est/1
  MOB_Estimator/2(y_mob_est) -> y_mob_est/1
  MOB_Estimator/3(vx_mob_est) -> vx_mob_est/1
  MOB_Estimator/4(vy_mob_est) -> vy_mob_est/1
  MOB_Estimator/5(track_age) -> track_age/1
  MOB_Estimator/6(track_valid) -> track_valid/1

== system USV_SAR_GNSS/State_Estimation/Navigation_Estimator ==
  x_gnss : Inport
  y_gnss : Inport  Port=2
  gnss_valid : Inport  Port=3
  MATLAB Function : MATLAB Function  TreatAsAtomicUnit=on
  x_nav : Outport
  y_nav : Outport  Port=2
  vx_nav : Outport  Port=3
  vy_nav : Outport  Port=4
  nav_age : Outport  Port=5
  nav_valid : Outport  Port=6
  wires:
  y_gnss/1 -> MATLAB Function/2(y_gnss)
  gnss_valid/1 -> MATLAB Function/3(gnss_valid)
  x_gnss/1 -> MATLAB Function/1(x_gnss)
  MATLAB Function/1(x_nav) -> x_nav/1
  MATLAB Function/2(y_nav) -> y_nav/1
  MATLAB Function/3(vx_nav) -> vx_nav/1
  MATLAB Function/4(vy_nav) -> vy_nav/1
  MATLAB Function/5(nav_age) -> nav_age/1
  MATLAB Function/6(nav_valid) -> nav_valid/1

== system USV_SAR_GNSS/Vehicle_Control/Heading_Controller ==
  psi_ref : Inport
  psi : Inport  Port=2
  r : Inport  Port=3
  Gain6 : Gain  Gain=Kp_heading
  Gain7 : Gain  Gain=Kd_heading
  Saturation : Saturate  UpperLimit=1  LowerLimit=0
  Sum4 : Sum  Inputs=|+-
  Sum5 : Sum  Inputs=|+-
  Trigonometric Function : Trigonometry
  Trigonometric Function1 : Trigonometry  Operator=cos
  Trigonometric Function2 : Trigonometry  Operator=atan2
  Trigonometric Function3 : Trigonometry  Operator=cos
  M_cmd : Outport
  heading_speed_factor : Outport  Port=2
  wires:
  Sum5/1 -> M_cmd/1
  psi_ref/1 -> Sum4/1
  r/1 -> Gain7/1
  Gain6/1 -> Sum5/1
  psi/1 -> Sum4/2
  Gain7/1 -> Sum5/2
  Sum4/1 -> Trigonometric Function/1, Trigonometric Function1/1
  Trigonometric Function/1 -> Trigonometric Function2/1
  Trigonometric Function1/1 -> Trigonometric Function2/2
  Trigonometric Function2/1 -> Trigonometric Function3/1, Gain6/1
  Trigonometric Function3/1 -> Saturation/1
  Saturation/1 -> heading_speed_factor/1

== system USV_SAR_GNSS/Vehicle_Control/Speed_Controller ==
  u_ref : Inport
  u : Inport  Port=2
  F_applied : Inport  Port=3
  Gain : Gain  Gain=K_aw
  Gain4 : Gain  Gain=Kp_u
  Gain5 : Gain  Gain=Ki_u
  Integrator5 : Integrator
  Sum : Sum  Inputs=|+-
  Sum1 : Sum  Inputs=|++
  Sum2 : Sum  Inputs=|+-
  Sum3 : Sum  Inputs=|++
  F_cmd : Outport
  wires:
  Integrator5/1 -> Gain5/1
  u_ref/1 -> Sum2/1
  u/1 -> Sum2/2
  Gain5/1 -> Sum3/2
  Sum2/1 -> Sum1/1, Gain4/1
  Gain4/1 -> Sum3/1
  Sum3/1 -> Sum/2, F_cmd/1
  F_applied/1 -> Sum/1
  Sum/1 -> Gain/1
  Sum1/1 -> Integrator5/1
  Gain/1 -> Sum1/2

== system USV_SAR_GNSS/Vehicle_Plant/USV_Dynamics ==
  F_cmd : Inport
  M_cmd : Inport  Port=2
  Gain : Gain  Gain=1/mass_usv
  Gain1 : Gain  Gain=drag_u
  Gain2 : Gain  Gain=1/inertia_z
  Gain3 : Gain  Gain=drag_r
  Integrator : Integrator
  Integrator2 : Integrator
  Sum : Sum  Inputs=|+-
  Sum1 : Sum  Inputs=|+-
  u : Outport
  r : Outport  Port=2
  wires:
  F_cmd/1 -> Sum/1
  Gain2/1 -> Integrator2/1
  Gain3/1 -> Sum1/2
  Integrator/1 -> Gain1/1, u/1  "u"
  Sum/1 -> Gain/1
  Gain/1 -> Integrator/1
  Gain1/1 -> Sum/2
  Sum1/1 -> Gain2/1
  Integrator2/1 -> Gain3/1, r/1  "r"
  M_cmd/1 -> Sum1/1

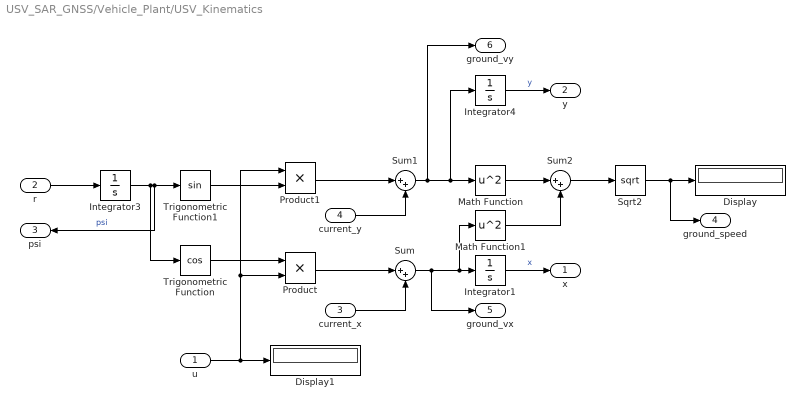
== system USV_SAR_GNSS/Vehicle_Plant/USV_Kinematics ==
  u : Inport
  r : Inport  Port=2
  current_x : Inport  Port=3
  current_y : Inport  Port=4
  Display : Display
  Display1 : Display
  Integrator1 : Integrator  InitialCondition=initial_x
  Integrator3 : Integrator  InitialCondition=initial_heading
  Integrator4 : Integrator  InitialCondition=initial_y
  Math Function : Math  Operator=square
  Math Function1 : Math  Operator=square
  Product : Product
  Product1 : Product
  Sqrt2 : Sqrt
  Sum : Sum  Inputs=|++
  Sum1 : Sum  Inputs=|++
  Sum2 : Sum  Inputs=|++
  Trigonometric Function : Trigonometry  Operator=cos
  Trigonometric Function1 : Trigonometry
  x : Outport
  y : Outport  Port=2
  psi : Outport  Port=3
  ground_speed : Outport  Port=4
  ground_vx : Outport  Port=5
  ground_vy : Outport  Port=6
  wires:
  Math Function/1 -> Sum2/1
  current_y/1 -> Sum1/2
  Integrator3/1 -> psi/1, Trigonometric Function1/1, Trigonometric Function/1  "psi"
  u/1 -> Product/2, Product1/1, Display1/1
  r/1 -> Integrator3/1
  Product/1 -> Sum/1
  Math Function1/1 -> Sum2/2
  Product1/1 -> Sum1/1
  Trigonometric Function/1 -> Product/1
  Trigonometric Function1/1 -> Product1/2
  current_x/1 -> Sum/2
  Sqrt2/1 -> Display/1, ground_speed/1
  Sum1/1 -> ground_vy/1, Math Function/1, Integrator4/1
  Sum2/1 -> Sqrt2/1
  Sum/1 -> ground_vx/1, Math Function1/1, Integrator1/1
  Integrator4/1 -> y/1  "y"
  Integrator1/1 -> x/1  "x"

== system USV_SAR_GNSS/Sensors/GNSS_Sensor/Valid_Position_Hold ==
  x_mesurement : Inport
  y_mesurement : Inport  Port=2
  Enable : EnablePort
  x_held : Outport
  y_held : Outport  Port=2
  wires:
  x_mesurement/1 -> x_held/1
  y_mesurement/1 -> y_held/1

== matlab function USV_SAR_GNSS/State_Estimation/Navigation_Estimator/MATLAB Function ==
  settings: updateMethod=DISCRETE  sampleTime=nav_sample_time
  data: x_gnss input; x_nav output; y_gnss input; gnss_valid input; y_nav output; vx_nav output; vy_nav output; nav_age output; nav_valid output; initial_x parameter; initial_y parameter; nav_sample_time parameter; gnss_sample_time parameter; nav_alpha parameter; nav_beta parameter; nav_max_prediction_time parameter
function [x_nav, y_nav, vx_nav, vy_nav, nav_age, nav_valid] = ...
    Alpha_Beta(x_gnss, y_gnss, gnss_valid, initial_x, initial_y, nav_sample_time, gnss_sample_time, nav_alpha, nav_beta, nav_max_prediction_time)

persistent px py vx vy contador tiempoSinMedida inicializado

% Inicialización al comenzar la simulación.
if isempty(contador)
    px = initial_x;
    py = initial_y;
    vx = 0;
    vy = 0;

    contador = 0;
    tiempoSinMedida = 0;
    inicializado = false;
else
    % Predicción entre medidas GNSS.
    px = px + vx * nav_sample_time;
    py = py + vy * nav_sample_time;

    tiempoSinMedida = tiempoSinMedida + nav_sample_time;
end

% Número de pasos del estimador entre muestras GNSS.
pasosGNSS = round(gnss_sample_time / nav_sample_time);

% Ambos relojes empiezan en t = 0.
nuevaMuestra = (contador == 0);

medidaValida = gnss_valid && ...
    isfinite(x_gnss) && isfinite(y_gnss);

if nuevaMuestra && medidaValida

    if ~inicializado
        % Primera posición válida: velocidad inicialmente desconocida.
        px = x_gnss;
        py = y_gnss;
        vx = 0;
        vy = 0;
        inicializado = true;
    else
        % Diferencia entre medida y predicción.
        errorX = x_gnss - px;
        errorY = y_gnss - py;

        intervalo = max(tiempoSinMedida, gnss_sample_time);

        % Corrección de posición.
        px = px + nav_alpha * errorX;
        py = py + nav_alpha * errorY;

        % Corrección de velocidad.
        vx = vx + (nav_beta / intervalo) * errorX;
        vy = vy + (nav_beta / intervalo) * errorY;
    end

    tiempoSinMedida = 0;
end

% Preparar el siguiente paso.
contador = contador + 1;

if contador >= pasosGNSS
    contador = 0;
end

% Salidas.
x_nav = px;
y_nav = py;
vx_nav = vx;
vy_nav = vy;
% Tiempo desde la última corrección GNSS válida.
nav_age = tiempoSinMedida;

% Permiso de uso según antigüedad de la estimación.
nav_valid = inicializado && ...
    (nav_age <= nav_max_prediction_time);
end

== matlab function USV_SAR_GNSS/State_Estimation/MOB_Tracking/MOB_Estimator ==
  settings: updateMethod=DISCRETE  sampleTime=mob_track_sample_time
  data: x_mob_meas input; x_mob_est output; y_mob_meas input; contact_valid input; y_mob_est output; vx_mob_est output; vy_mob_est output; track_age output; track_valid output; mob_track_sample_time parameter; mob_track_alpha parameter; mob_track_beta parameter; mob_track_max_age parameter
function [x_mob_est, y_mob_est, vx_mob_est, vy_mob_est, ...
    track_age, track_valid] = ...
    MOB_Estimator(x_mob_meas, y_mob_meas, contact_valid, mob_track_sample_time, mob_track_alpha, mob_track_beta, mob_track_max_age)

persistent px py vx vy age initialized

% Inicialización al comenzar la simulación.
if isempty(initialized)
    px = 0;
    py = 0;
    vx = 0;
    vy = 0;

    age = inf;
    initialized = false;

else
    % Predicción entre observaciones.
    if initialized
        px = px + vx * mob_track_sample_time;
        py = py + vy * mob_track_sample_time;

        age = age + mob_track_sample_time;
    end
end

% Comprobar si la observación puede utilizarse.
measurement_valid = contact_valid && ...
    isfinite(x_mob_meas) && isfinite(y_mob_meas);

if measurement_valid

    if ~initialized
        % Primera observación válida.
        px = x_mob_meas;
        py = y_mob_meas;

        vx = 0;
        vy = 0;

        initialized = true;

    else
        % Diferencia entre observación y predicción.
        error_x = x_mob_meas - px;
        error_y = y_mob_meas - py;

        interval = max(age, mob_track_sample_time);

        % Corrección de posición.
        px = px + mob_track_alpha * error_x;
        py = py + mob_track_alpha * error_y;

        % Corrección de velocidad.
        vx = vx + (mob_track_beta / interval) * error_x;
        vy = vy + (mob_track_beta / interval) * error_y;
    end

    age = 0;
end

% Salidas.
x_mob_est = px;
y_mob_est = py;

vx_mob_est = vx;
vy_mob_est = vy;

track_age = age;

track_valid = initialized && ...
    (age <= mob_track_max_age);

end
